simulink model "dual_thyristor_bridge_rectifier"  (R2025b)
settings: Solver=ode1be  StartTime=0.0  StopTime=simlength  FixedStep=tc  MaxStep=tc
values from neighbouring files (symbols this model uses):
  n1 = 35    [voltage_spectrum_analysis.m]
  omega_grid_emulator_nom = w_grid    (= 314.159265359)    [grid_emulator.m]
  vn_eta_pu = 0    [grid_emulator.m]
  vn_xi_pu = 0    [grid_emulator.m]
  vp_xi_pu = 1    [grid_emulator.m]
  w_grid = f_grid*2*pi    (= 314.159265359)    [grid_emulator.m]
undefined symbols (not defined in the file or in its folder): CSF_11, CSF_13, CSF_5, CSF_7, delta_fht1, Idc_traction_normalization_factor, ki_u_ctrl, kp_u_ctrl, Ld_fht1, LFu_dc, LSF_11, LSF_13, LSF_5, LSF_7, magnitude, n10, omega_fht1, pll_i1, pll_p, RLFu_dc, tc, Tcontrol_rect, ts_ctrl_rect, ugrid_factor, Vdc_traction_normalization_factor, Vgrid_phase_normalization_factor
libraries: fl_lib x299, nesl_utility x67, ee_lib x24, single_phase_transformer_lib x3, cstblocks x3
(part 1 of 6)
settings Model: SimulationMode=accelerator  Creator=dbagn  LastModifiedBy=ltnbda
settings SolverCC: NumberNewtonIterations=3.0  ZeroCrossControl=DisableAll  AlgebraicLoopSolver=TrustRegion  SolverResetMethod=Robust
settings DataIOCC: SaveOutput=off  SignalLogging=off  DSMLogging=off  SaveTime=off  ReturnWorkspaceOutputs=off
settings OptimizationCC: ReuseModelBlockBuffer=off  SimCompilerOptimization=on
settings DebuggingCC: UnconnectedInputMsg=warning  UnconnectedOutputMsg=warning  UnconnectedLineMsg=warning
settings ModelReferenceCC: EnableRefExpFcnMdlSchedulingChecks=on
settings SFSimCC: CustomCodeUndefinedFunction=ThrowError
settings SFSimCC: SimCustomHeaderCode=|
  | #include "math_f.h"
  | #include "mavgflt.h"
  | #include "mavgflt_simulink.h"
  | #include "bemf_obsv.h"
  | #include "bemf_obsv_simulink.h"
  | #include "bemf_obsv_load_est.h"
  | #include "bemf_obsv_load_est_simulink.h"
  | #include "dqvector_pi.h"
  | #include "dqvector_pi_simulink.h"
  | #include "sv_pwm_simulink.h"
  | #include "sv_pwm.h"
  | #include "twelve_pulse_rect.h"
  | #include "first_harmonic_tracker.h"
  | #include "first_harmonic_tracker_simulink.h"
  | #include "dqpll_thyr.h"
  | #include "dqpll_thyr_simulink.h"
  | #include "dqpll_grid.h"
  | #include "dqpll_grid_simulink.h"
settings SFSimCC: SimUserSources=|
  | "mavgflt_simulink.c"
  | "mavgflt.c"
  | "bemf_obsv_simulink.c"
  | "bemf_obsv.c"
  | "bemf_obsv_load_est_simulink.c"
  | "bemf_obsv_load_est.c"
  | "dqvector_pi.c"
  | "dqvector_pi_simulink.c"
  | "sv_pwm_simulink.c"
  | "sv_pwm.c"
  | "twelve_pulse_rect.c"
  | "first_harmonic_tracker_simulink.c"
  | "first_harmonic_tracker.c"
  | "dqpll_thyr_simulink.c"
  | "dqpll_thyr.c"
  | "dqpll_grid_simulink.c"
  | "dqpll_grid.c"
settings SFSimCC: SimUserIncludeDirs=|
  | include
  | src
settings RTWCC: GPUComputeCapability=3.5  DLArmComputeVersion=19.05

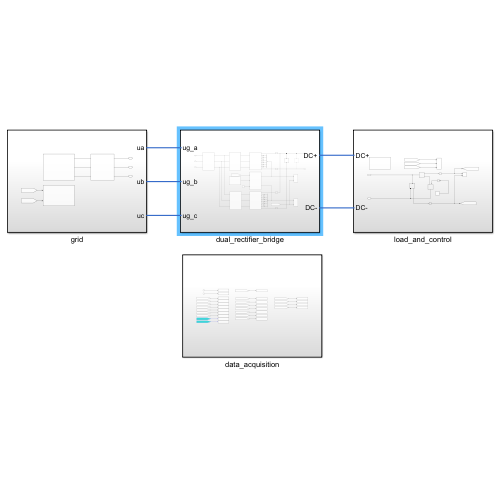
[thumbnail: Simulink's stored preview of the top-level diagram]
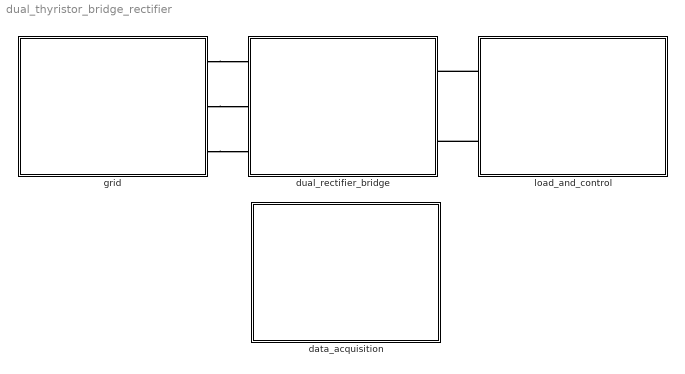
== system dual_thyristor_bridge_rectifier ==
  data_acquisition : Subsystem
  dual_rectifier_bridge : Subsystem
  grid : Subsystem
  load_and_control : Subsystem
  connections:
  grid/RConn1 -- dual_rectifier_bridge/LConn1
  grid/RConn2 -- dual_rectifier_bridge/LConn2
  grid/RConn3 -- dual_rectifier_bridge/LConn3
  load_and_control/LConn1 -- dual_rectifier_bridge/RConn1
  load_and_control/LConn2 -- dual_rectifier_bridge/RConn2

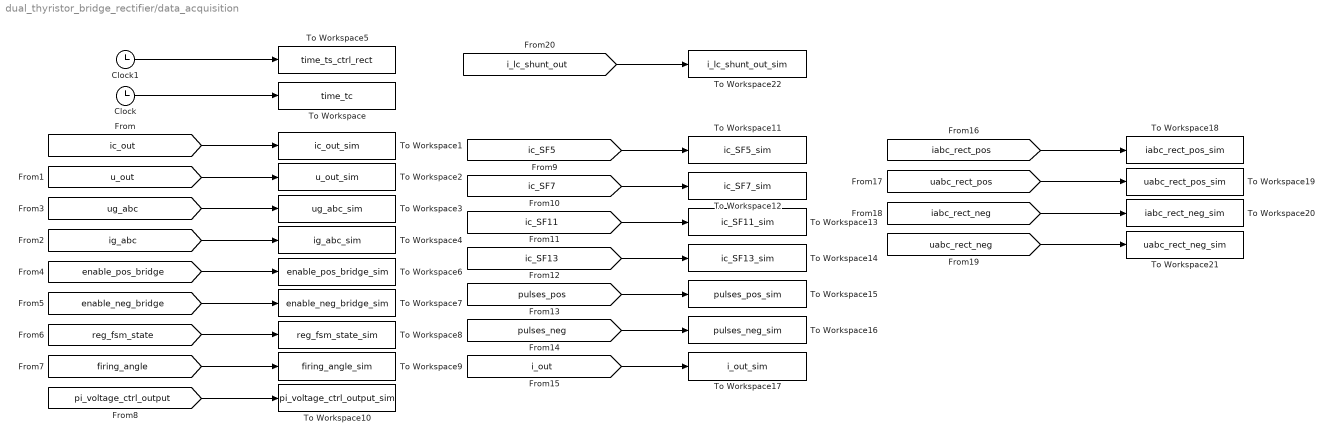
== system dual_thyristor_bridge_rectifier/data_acquisition ==
  Clock : Clock
  Clock1 : Clock
  To Workspace : ToWorkspace  VariableName=time_tc  SaveFormat=Timeseries  SampleTime=tc
      settings: MaxDataPoints=Nc
  To Workspace1 : ToWorkspace  VariableName=ic_out_sim  SaveFormat=Timeseries  SampleTime=tc
      settings: MaxDataPoints=Nc
  To Workspace10 : ToWorkspace  VariableName=pi_voltage_ctrl_output_sim  SaveFormat=Timeseries  SampleTime=ts_ctrl_rect
      settings: MaxDataPoints=Ns_ctrl_rect
  To Workspace11 : ToWorkspace  VariableName=ic_SF5_sim  SaveFormat=Timeseries  SampleTime=tc
      settings: MaxDataPoints=Nc
  To Workspace12 : ToWorkspace  VariableName=ic_SF7_sim  SaveFormat=Timeseries  SampleTime=tc
      settings: MaxDataPoints=Nc
  To Workspace13 : ToWorkspace  VariableName=ic_SF11_sim  SaveFormat=Timeseries  SampleTime=tc
      settings: MaxDataPoints=Nc
  To Workspace14 : ToWorkspace  VariableName=ic_SF13_sim  SaveFormat=Timeseries  SampleTime=tc
      settings: MaxDataPoints=Nc
  To Workspace15 : ToWorkspace  VariableName=pulses_pos_sim  SaveFormat=Timeseries  SampleTime=tc
      settings: MaxDataPoints=Nc
  To Workspace16 : ToWorkspace  VariableName=pulses_neg_sim  SaveFormat=Timeseries  SampleTime=tc
      settings: MaxDataPoints=Nc
  To Workspace17 : ToWorkspace  VariableName=i_out_sim  SaveFormat=Timeseries  SampleTime=tc
      settings: MaxDataPoints=Nc
  To Workspace18 : ToWorkspace  VariableName=iabc_rect_pos_sim  SaveFormat=Timeseries  SampleTime=tc
      settings: MaxDataPoints=Nc
  To Workspace19 : ToWorkspace  VariableName=uabc_rect_pos_sim  SaveFormat=Timeseries  SampleTime=tc
      settings: MaxDataPoints=Nc
  To Workspace2 : ToWorkspace  VariableName=u_out_sim  SaveFormat=Timeseries  SampleTime=tc
      settings: MaxDataPoints=Nc
  To Workspace20 : ToWorkspace  VariableName=iabc_rect_neg_sim  SaveFormat=Timeseries  SampleTime=tc
      settings: MaxDataPoints=Nc
  To Workspace21 : ToWorkspace  VariableName=uabc_rect_neg_sim  SaveFormat=Timeseries  SampleTime=tc
      settings: MaxDataPoints=Nc
  To Workspace22 : ToWorkspace  VariableName=i_lc_shunt_out_sim  SaveFormat=Timeseries  SampleTime=tc
      settings: MaxDataPoints=Nc
  To Workspace3 : ToWorkspace  VariableName=ug_abc_sim  SaveFormat=Timeseries  SampleTime=tc
      settings: MaxDataPoints=Nc
  To Workspace4 : ToWorkspace  VariableName=ig_abc_sim  SaveFormat=Timeseries  SampleTime=tc
      settings: MaxDataPoints=Nc
  To Workspace5 : ToWorkspace  VariableName=time_ts_ctrl_rect  SaveFormat=Timeseries  SampleTime=tc
      settings: MaxDataPoints=Nc
  To Workspace6 : ToWorkspace  VariableName=enable_pos_bridge_sim  SaveFormat=Timeseries  SampleTime=ts_ctrl_rect
      settings: MaxDataPoints=Ns_ctrl_rect
  To Workspace7 : ToWorkspace  VariableName=enable_neg_bridge_sim  SaveFormat=Timeseries  SampleTime=ts_ctrl_rect
      settings: MaxDataPoints=Ns_ctrl_rect
  To Workspace8 : ToWorkspace  VariableName=reg_fsm_state_sim  SaveFormat=Timeseries  SampleTime=ts_ctrl_rect
      settings: MaxDataPoints=Ns_ctrl_rect
  To Workspace9 : ToWorkspace  VariableName=firing_angle_sim  SaveFormat=Timeseries  SampleTime=ts_ctrl_rect
      settings: MaxDataPoints=Ns_ctrl_rect
  wires:
  [ic_out] -> To Workspace1/1
  Clock/1 -> To Workspace/1
  [ug_abc] -> To Workspace3/1
  [ig_abc] -> To Workspace4/1
  [u_out] -> To Workspace2/1
  Clock1/1 -> To Workspace5/1
  [enable_pos_bridge] -> To Workspace6/1
  [enable_neg_bridge] -> To Workspace7/1
  [reg_fsm_state] -> To Workspace8/1
  [firing_angle] -> To Workspace9/1
  [pi_voltage_ctrl_output] -> To Workspace10/1
  [ic_SF5] -> To Workspace11/1
  [ic_SF7] -> To Workspace12/1
  [ic_SF11] -> To Workspace13/1
  [ic_SF13] -> To Workspace14/1
  [pulses_pos] -> To Workspace15/1
  [pulses_neg] -> To Workspace16/1
  [i_out] -> To Workspace17/1
  [iabc_rect_pos] -> To Workspace18/1
  [uabc_rect_pos] -> To Workspace19/1
  [uabc_rect_neg] -> To Workspace21/1
  [iabc_rect_neg] -> To Workspace20/1
  [i_lc_shunt_out] -> To Workspace22/1

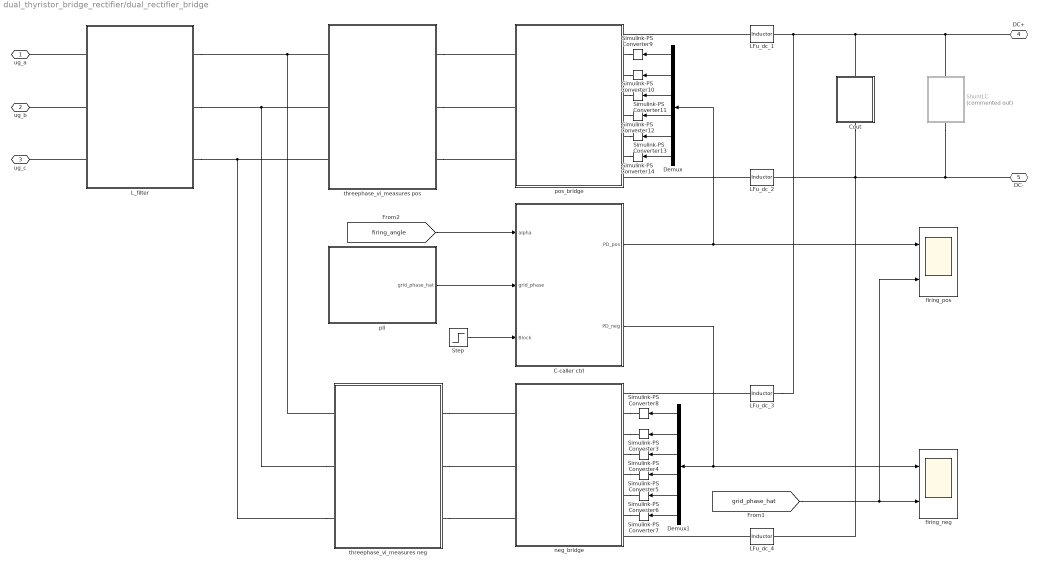
== system dual_thyristor_bridge_rectifier/dual_rectifier_bridge ==
  C-caller ctrl : Subsystem
  Cout : Subsystem
  Demux : Demux  Outputs=6
  Demux1 : Demux  Outputs=6
  LFu_dc_{1..4} (4 alike) : fl_lib/Electrical/Electrical Elements/Inductor  l=LFu_dc/2 H  r=RLFu_dc/2 Ohm  g=1e-9 1/Ohm  i_specify=off  i_priority=None  i=0 A  i_nominal_specify=off  i_nominal_value=1  i_nominal_unit=A  v_specify=off  v_priority=None  v=0 V  v_nominal_specify=off  v_nominal_value=1  v_nominal_unit=V  i_L_specify=off  i_L_priority=High  i_L=0 A  i_L_nominal_specify=off  i_L_nominal_value=1  i_L_nominal_unit=A
  L_filter : Subsystem
  ShuntLC : Subsystem  Commented=on
  Simulink-PS Converter{3,5..10,12..14} (10 alike) : nesl_utility/Simulink-PS Converter  PhysicalDomain=network_engine_domain  SubClassName=ps_input  LeftPortType=input  RightPortType=output  PseudoPeriodic=off  Frequencies=[]  NoiseDistribution=none  NoiseParameters=[]  Unit=V  AffineConversion=on  FilteringAndDerivatives=provide  SimscapeFilterOrder=1  InputFilterTimeConstant=0.001  UdotUserProvided=0
  Simulink-PS Converter11 : nesl_utility/Simulink-PS Converter  PhysicalDomain=network_engine_domain  SubClassName=ps_input  LeftPortType=input  RightPortType=output  PseudoPeriodic=off  Frequencies=[]  NoiseDistribution=none  NoiseParameters=[]  Unit=V  AffineConversion=off  FilteringAndDerivatives=provide  SimscapeFilterOrder=1  InputFilterTimeConstant=0.001  UdotUserProvided=0
  Simulink-PS Converter4 : nesl_utility/Simulink-PS Converter  PhysicalDomain=network_engine_domain  SubClassName=ps_input  LeftPortType=input  RightPortType=output  PseudoPeriodic=off  Frequencies=[]  NoiseDistribution=none  NoiseParameters=[]  Unit=V  AffineConversion=off  FilteringAndDerivatives=provide  SimscapeFilterOrder=1  InputFilterTimeConstant=0.001  UdotUserProvided=0
  Step : Step  Time=0  Before=1  After=0
  firing_neg : Scope  NumInputPorts=2
      settings: SampleTime=ts  ActiveDisplayYMinimum=-1.5  ActiveDisplayYMaximum=13.5
  firing_pos : Scope  NumInputPorts=2
      settings: SampleTime=ts  ActiveDisplayYMinimum=-1.5  ActiveDisplayYMaximum=13.5
  neg_bridge : Subsystem
  pll : Subsystem
  pos_bridge : Subsystem
  threephase_vi_measures neg : Subsystem
  threephase_vi_measures pos : Subsystem
  ug_a : PMIOPort  Side=Left
  ug_b : PMIOPort  Port=2  Side=Left
  ug_c : PMIOPort  Port=3  Side=Left
  DC+ : PMIOPort  Port=4  Side=Right
  DC- : PMIOPort  Port=5  Side=Right
  wires:
  Demux1/1 -> Simulink-PS Converter8/1
  Step/1 -> C-caller ctrl/3(Block)
  C-caller ctrl/1(PD_pos) -> firing_pos/1, Demux/1
  Demux/6 -> Simulink-PS Converter14/1
  Demux1/4 -> Simulink-PS Converter5/1
  Demux1/6 -> Simulink-PS Converter7/1
  [firing_angle] -> C-caller ctrl/1(alpha)
  Demux1/3 -> Simulink-PS Converter4/1
  Demux/4 -> Simulink-PS Converter12/1
  pll/1(grid_phase_hat) -> C-caller ctrl/2(grid_phase)
  C-caller ctrl/2(PD_neg) -> firing_neg/1, Demux1/1
  Demux1/2 -> Simulink-PS Converter3/1
  Demux/1 -> Simulink-PS Converter9/1
  Demux/2 -> Simulink-PS Converter10/1
  Demux/3 -> Simulink-PS Converter11/1
  Demux1/5 -> Simulink-PS Converter6/1
  Demux/5 -> Simulink-PS Converter13/1
  [grid_phase_hat] -> firing_neg/2, firing_pos/2
  connections:
  L_filter/RConn1 -- ug_a/RConn1
  L_filter/RConn2 -- ug_b/RConn1
  L_filter/RConn3 -- ug_c/RConn1
  pos_bridge/LConn3 -- Simulink-PS Converter10/RConn1
  neg_bridge/LConn6 -- Simulink-PS Converter6/RConn1
  neg_bridge/LConn5 -- Simulink-PS Converter5/RConn1
  pos_bridge/LConn5 -- Simulink-PS Converter12/RConn1
  neg_bridge/LConn2 -- Simulink-PS Converter8/RConn1
  pos_bridge/LConn2 -- Simulink-PS Converter9/RConn1
  neg_bridge/LConn3 -- Simulink-PS Converter3/RConn1
  pos_bridge/LConn4 -- Simulink-PS Converter11/RConn1
  neg_bridge/LConn7 -- Simulink-PS Converter7/RConn1
  pos_bridge/LConn6 -- Simulink-PS Converter13/RConn1
  pos_bridge/LConn7 -- Simulink-PS Converter14/RConn1
  neg_bridge/LConn4 -- Simulink-PS Converter4/RConn1
  threephase_vi_measures neg/LConn2 -- L_filter/LConn2 -- threephase_vi_measures pos/LConn2
  L_filter/LConn1 -- threephase_vi_measures neg/LConn1 -- threephase_vi_measures pos/LConn1
  threephase_vi_measures neg/LConn3 -- L_filter/LConn3 -- threephase_vi_measures pos/LConn3
  threephase_vi_measures pos/RConn1 -- pos_bridge/RConn1
  threephase_vi_measures pos/RConn2 -- pos_bridge/RConn2
  threephase_vi_measures pos/RConn3 -- pos_bridge/RConn3
  threephase_vi_measures neg/RConn1 -- neg_bridge/RConn1
  threephase_vi_measures neg/RConn2 -- neg_bridge/RConn2
  threephase_vi_measures neg/RConn3 -- neg_bridge/RConn3
  LFu_dc_4/RConn1 -- LFu_dc_2/RConn1 -- Cout/RConn1 -- ShuntLC/RConn1 -- DC-/RConn1
  LFu_dc_1/RConn1 -- LFu_dc_3/RConn1 -- Cout/LConn1 -- ShuntLC/LConn1 -- DC+/RConn1
  LFu_dc_1/LConn1 -- pos_bridge/LConn1
  LFu_dc_2/LConn1 -- pos_bridge/LConn8
  neg_bridge/LConn1 -- LFu_dc_3/LConn1
  LFu_dc_4/LConn1 -- neg_bridge/LConn8

== system dual_thyristor_bridge_rectifier/grid ==
  grid_emulator : Subsystem
  instantaneus_power : Subsystem
  threephase_vi_measures : Subsystem
  ua : PMIOPort  Side=Right
  ub : PMIOPort  Port=2  Side=Right
  uc : PMIOPort  Port=3  Side=Right
  wires:
  [ug_abc] -> instantaneus_power/1(Vline)
  [ig_abc] -> instantaneus_power/2(Iline)
  connections:
  threephase_vi_measures/LConn3 -- grid_emulator/RConn3
  threephase_vi_measures/LConn1 -- grid_emulator/RConn1
  threephase_vi_measures/RConn2 -- ub/RConn1
  threephase_vi_measures/LConn2 -- grid_emulator/RConn2
  threephase_vi_measures/RConn1 -- ua/RConn1
  threephase_vi_measures/RConn3 -- uc/RConn1

== system dual_thyristor_bridge_rectifier/load_and_control ==
  Controlled Current Source : fl_lib/Electrical/Electrical Sources/Controlled Current Source
  Current Sensor : fl_lib/Electrical/Electrical Sensors/Current Sensor
  PS-Simulink Converter : nesl_utility/PS-Simulink Converter  PhysicalDomain=network_engine_domain  SubClassName=ps_output  LeftPortType=input  RightPortType=output  PseudoPeriodic=off  Frequencies=[]  VectorFormat=1-D array  Unit=A  AffineConversion=off
  PS-Simulink Converter1 : nesl_utility/PS-Simulink Converter  PhysicalDomain=network_engine_domain  SubClassName=ps_output  LeftPortType=input  RightPortType=output  PseudoPeriodic=off  Frequencies=[]  VectorFormat=1-D array  Unit=V  AffineConversion=on
  Simulink-PS Converter : nesl_utility/Simulink-PS Converter  PhysicalDomain=network_engine_domain  SubClassName=ps_input  LeftPortType=input  RightPortType=output  PseudoPeriodic=off  Frequencies=[]  NoiseDistribution=none  NoiseParameters=[]  Unit=1  AffineConversion=off  FilteringAndDerivatives=provide  SimscapeFilterOrder=1  InputFilterTimeConstant=0.001  UdotUserProvided=0
  Sine Wave : Sin  Amplitude=Idc_traction_normalization_factor  Frequency=pi/2  SampleTime=0
  Voltage Sensor : fl_lib/Electrical/Electrical Sensors/Voltage Sensor
  controller : Subsystem
  iu_out : Scope  NumInputPorts=2
      settings: SampleTime=ts  ActiveDisplayYMinimum=-2016.1290322580644  ActiveDisplayYMaximum=2016.1290322580644  DataLoggingVariableName=ScopeData3
  ui_Cout : Scope  NumInputPorts=3
      settings: SampleTime=ts  ActiveDisplayYMinimum=-646.93724  ActiveDisplayYMaximum=1108.66938
  DC+ : PMIOPort  Side=Left
  DC- : PMIOPort  Port=2  Side=Left
  tag scope: i_out=global, u_out=global
  wires:
  PS-Simulink Converter/1 -> [i_out], iu_out/1  "i_out"
  PS-Simulink Converter1/1 -> [u_out], iu_out/2  "u_out"
  Sine Wave/1 -> Simulink-PS Converter/1
  [u_out] -> ui_Cout/2  "u_out"
  [ic_out] -> ui_Cout/1  "ic_out"
  [i_lc_shunt_out] -> ui_Cout/3  "i_lc_shunt_out"
  connections:
  Voltage Sensor/RConn1 -- PS-Simulink Converter1/LConn1
  DC+/RConn1 -- Current Sensor/LConn1 -- Voltage Sensor/LConn1
  Simulink-PS Converter/RConn1 -- Controlled Current Source/RConn1
  Current Sensor/RConn2 -- Controlled Current Source/RConn2
  PS-Simulink Converter/LConn1 -- Current Sensor/RConn1
  DC-/RConn1 -- Controlled Current Source/LConn1 -- Voltage Sensor/RConn2

== system dual_thyristor_bridge_rectifier/dual_rectifier_bridge/C-caller ctrl ==
  alpha : Inport
  grid_phase : Inport  Port=2
  Block : Inport  Port=3
  C Caller : CCaller  FunctionName=twvprProcessSimulink  PortSpecificationStruct="%)30     .    R @   8    (     @         %    \"     4    !     0         %  0 \"0    $    _    07)G3F%M90  4&]R=$YA;64 4V-O<&4     26YD97@     5'EP90      4VEZ90      27-';&]B86P   X    P    !@    @    $          4    (     0    (    !         !   @!W=   #@   #     &    \"     0         !0    @    !     @    $         $  \" '=T   .    .     8    (    !          %    \"     $    %     0         0  ...(+2649 chars)"  SampleTime=ts_ctrl_rect
  Constant : Constant  Value=[0 0 0 0 0 0]
  Data Type Conversion1 : DataTypeConversion  OutDataTypeStr=single  SaturateOnIntegerOverflow=off  RndMeth=Floor
  Data Type Conversion2 : DataTypeConversion  OutDataTypeStr=single  SaturateOnIntegerOverflow=off  RndMeth=Floor
  Data Type Conversion4 : DataTypeConversion  OutDataTypeStr=int32  SaturateOnIntegerOverflow=off  RndMeth=Floor
  Subsystem2 : Subsystem
  Subsystem3 : Subsystem
  Zero-Order Hold1 : ZeroOrderHold  SampleTime=ts_ctrl_rect
  Zero-Order Hold2 : ZeroOrderHold  SampleTime=ts_ctrl_rect
  Zero-Order Hold3 : ZeroOrderHold  SampleTime=ts_ctrl_rect
  neg : Switch  Criteria=u2 > Threshold  Threshold=0.5  SaturateOnIntegerOverflow=off  InputSameDT=off
  pos : Switch  Criteria=u2 > Threshold  Threshold=0.5  SaturateOnIntegerOverflow=off  InputSameDT=off
  PD_pos : Outport  InitialOutput=0  VectorParamsAs1DForOutWhenUnconnected=off
  PD_neg : Outport  Port=2  InitialOutput=0  VectorParamsAs1DForOutWhenUnconnected=off
  tag scope: pulses_neg=global, pulses_pos=global
  wires:
  alpha/1 -> Data Type Conversion2/1
  grid_phase/1 -> Data Type Conversion1/1
  Data Type Conversion2/1 -> Zero-Order Hold2/1
  Data Type Conversion1/1 -> Zero-Order Hold3/1
  Data Type Conversion4/1 -> Zero-Order Hold1/1
  Block/1 -> Data Type Conversion4/1
  C Caller/1 -> Subsystem3/1("PY ")
  C Caller/2 -> Subsystem2/1("PD ")
  Constant/1 -> pos/3, neg/3
  Subsystem2/1(PD) -> neg/1, pos/1
  [enable_pos_bridge] -> pos/2
  [enable_neg_bridge] -> neg/2
  pos/1 -> [pulses_pos], PD_pos/1
  neg/1 -> [pulses_neg], PD_neg/1
  Zero-Order Hold3/1 -> C Caller/1
  Zero-Order Hold2/1 -> C Caller/2
  Zero-Order Hold1/1 -> C Caller/3

== system dual_thyristor_bridge_rectifier/dual_rectifier_bridge/Cout ==
  Capacitor : fl_lib/Electrical/Electrical Elements/Capacitor  c=CFu_dc F  r=RCFu_dc Ohm  g=0 1/Ohm  i_specify=off  i_priority=None  i=0 A  i_nominal_specify=off  i_nominal_value=1  i_nominal_unit=A  v_specify=off  v_priority=None  v=0 V  v_nominal_specify=off  v_nominal_value=1  v_nominal_unit=V  vc_specify=off  vc_priority=High  vc=0 V  vc_nominal_specify=off  vc_nominal_value=1  vc_nominal_unit=V
  Current Sensor1 : fl_lib/Electrical/Electrical Sensors/Current Sensor
  PS-Simulink Converter2 : nesl_utility/PS-Simulink Converter  PhysicalDomain=network_engine_domain  SubClassName=ps_output  LeftPortType=input  RightPortType=output  PseudoPeriodic=off  Frequencies=[]  VectorFormat=1-D array  Unit=A  AffineConversion=off
  u+ : PMIOPort  Side=Left
  u- : PMIOPort  Port=2  Side=Right
  tag scope: ic_out=global
  wires:
  PS-Simulink Converter2/1 -> [ic_out]
  connections:
  Capacitor/RConn1 -- u-/RConn1
  Current Sensor1/RConn2 -- Capacitor/LConn1
  PS-Simulink Converter2/LConn1 -- Current Sensor1/RConn1
  Current Sensor1/LConn1 -- u+/RConn1

== system dual_thyristor_bridge_rectifier/dual_rectifier_bridge/L_filter ==
  Inductor : fl_lib/Electrical/Electrical Elements/Inductor  l=1e-6 H  r=0 Ohm  g=1e-9 1/Ohm  i_specify=on  i_priority=High  i=0 A  i_nominal_specify=off  i_nominal_value=1  i_nominal_unit=A  v_specify=off  v_priority=None  v=0 V  v_nominal_specify=off  v_nominal_value=1  v_nominal_unit=V  i_L_specify=off  i_L_priority=High  i_L=0 A  i_L_nominal_specify=off  i_L_nominal_value=1  i_L_nominal_unit=A
  Inductor1 : fl_lib/Electrical/Electrical Elements/Inductor  l=1e-6 H  r=0 Ohm  g=1e-9 1/Ohm  i_specify=on  i_priority=High  i=0 A  i_nominal_specify=off  i_nominal_value=1  i_nominal_unit=A  v_specify=off  v_priority=None  v=0 V  v_nominal_specify=off  v_nominal_value=1  v_nominal_unit=V  i_L_specify=off  i_L_priority=High  i_L=0 A  i_L_nominal_specify=off  i_L_nominal_value=1  i_L_nominal_unit=A
  Inductor2 : fl_lib/Electrical/Electrical Elements/Inductor  l=1e-6 H  r=0 Ohm  g=1e-9 1/Ohm  i_specify=on  i_priority=High  i=0 A  i_nominal_specify=off  i_nominal_value=1  i_nominal_unit=A  v_specify=off  v_priority=None  v=0 V  v_nominal_specify=off  v_nominal_value=1  v_nominal_unit=V  i_L_specify=off  i_L_priority=High  i_L=0 A  i_L_nominal_specify=off  i_L_nominal_value=1  i_L_nominal_unit=A
  i_SFs : Scope  NumInputPorts=4
      settings: SampleTime=tc  ActiveDisplayYMinimum=-334.41525  ActiveDisplayYMaximum=336.06574  DataLoggingVariableName=ScopeData2
  shunt_passive_filter_11 : Subsystem  mask{CSF=CSF_11, LSF=LSF_11, RCSF=5e-3}
      mask prompts: CSF "Shunt Capacitor"; LSF "Shunt Inductor"; RCSF "Shunt Resistor"
      mask Display: disp('SPF');
  shunt_passive_filter_13 : Subsystem  mask{CSF=CSF_13, LSF=LSF_13, RCSF=5e-3}
      mask prompts: CSF "Shunt Capacitor"; LSF "Shunt Inductor"; RCSF "Shunt Resistor"
      mask Display: disp('SPF');
  shunt_passive_filter_5 : Subsystem  mask{CSF=CSF_5, LSF=LSF_5, RCSF=5e-3}
      mask prompts: CSF "Shunt Capacitor"; LSF "Shunt Inductor"; RCSF "Shunt Resistor"
      mask Display: disp('SPF');
  shunt_passive_filter_7 : Subsystem  mask{CSF=CSF_7, LSF=LSF_7, RCSF=5e-3}
      mask prompts: CSF "Shunt Capacitor"; LSF "Shunt Inductor"; RCSF "Shunt Resistor"
      mask Display: disp('SPF');
  ui_measure : Subsystem
  us_a : PMIOPort  Side=Left
  ug_a : PMIOPort  Port=2  Side=Right
  us_b : PMIOPort  Port=3  Side=Left
  ug_b : PMIOPort  Port=4  Side=Right
  us_c : PMIOPort  Port=5  Side=Left
  ug_c : PMIOPort  Port=6  Side=Right
  wires:
  [ic_SF5] -> i_SFs/1
  [ic_SF7] -> i_SFs/2
  [ic_SF11] -> i_SFs/3
  [ic_SF13] -> i_SFs/4
  connections:
  ui_measure/RConn1 -- shunt_passive_filter_7/RConn1 -- shunt_passive_filter_11/RConn1 -- shunt_passive_filter_13/RConn1 -- Inductor/LConn1 -- shunt_passive_filter_5/RConn1
  ui_measure/RConn2 -- shunt_passive_filter_7/RConn2 -- shunt_passive_filter_11/RConn2 -- shunt_passive_filter_13/RConn2 -- Inductor1/LConn1 -- shunt_passive_filter_5/RConn2
  ui_measure/RConn3 -- shunt_passive_filter_7/RConn3 -- shunt_passive_filter_11/RConn3 -- shunt_passive_filter_13/RConn3 -- Inductor2/LConn1 -- shunt_passive_filter_5/RConn3
  us_a/RConn1 -- Inductor/RConn1
  Inductor1/RConn1 -- us_b/RConn1
  Inductor2/RConn1 -- us_c/RConn1
  ug_b/RConn1 -- ui_measure/LConn2
  ug_a/RConn1 -- ui_measure/LConn1
  ug_c/RConn1 -- ui_measure/LConn3

== system dual_thyristor_bridge_rectifier/dual_rectifier_bridge/ShuntLC ==
  Capacitor : fl_lib/Electrical/Electrical Elements/Capacitor  c=C_shunt_dc F  r=RC_shunt_dc Ohm  g=0 1/Ohm  i_specify=off  i_priority=None  i=0 A  i_nominal_specify=off  i_nominal_value=1  i_nominal_unit=A  v_specify=off  v_priority=None  v=0 V  v_nominal_specify=off  v_nominal_value=1  v_nominal_unit=V  vc_specify=off  vc_priority=High  vc=0 V  vc_nominal_specify=off  vc_nominal_value=1  vc_nominal_unit=V
  Capacitor1 : fl_lib/Electrical/Electrical Elements/Capacitor  c=C_shunt_dc F  r=RC_shunt_dc Ohm  g=0 1/Ohm  i_specify=off  i_priority=None  i=0 A  i_nominal_specify=off  i_nominal_value=1  i_nominal_unit=A  v_specify=off  v_priority=None  v=0 V  v_nominal_specify=off  v_nominal_value=1  v_nominal_unit=V  vc_specify=off  vc_priority=High  vc=0 V  vc_nominal_specify=off  vc_nominal_value=1  vc_nominal_unit=V
  Current Sensor1 : fl_lib/Electrical/Electrical Sensors/Current Sensor
  Inductor : fl_lib/Electrical/Electrical Elements/Inductor  l=L_shunt_dc H  r=0 Ohm  g=1e-9 1/Ohm  i_specify=off  i_priority=None  i=0 A  i_nominal_specify=off  i_nominal_value=1  i_nominal_unit=A  v_specify=off  v_priority=None  v=0 V  v_nominal_specify=off  v_nominal_value=1  v_nominal_unit=V  i_L_specify=off  i_L_priority=High  i_L=0 A  i_L_nominal_specify=off  i_L_nominal_value=1  i_L_nominal_unit=A
  PS-Simulink Converter2 : nesl_utility/PS-Simulink Converter  PhysicalDomain=network_engine_domain  SubClassName=ps_output  LeftPortType=input  RightPortType=output  PseudoPeriodic=off  Frequencies=[]  VectorFormat=1-D array  Unit=A  AffineConversion=off
  u+ : PMIOPort  Side=Left
  u- : PMIOPort  Port=2  Side=Right
  tag scope: i_lc_shunt_out=global
  wires:
  PS-Simulink Converter2/1 -> [i_lc_shunt_out]
  connections:
  Current Sensor1/LConn1 -- u+/RConn1
  PS-Simulink Converter2/LConn1 -- Current Sensor1/RConn1
  Current Sensor1/RConn2 -- Capacitor1/LConn1 -- Capacitor/LConn1
  Capacitor/RConn1 -- Capacitor1/RConn1 -- Inductor/LConn1
  Inductor/RConn1 -- u-/RConn1

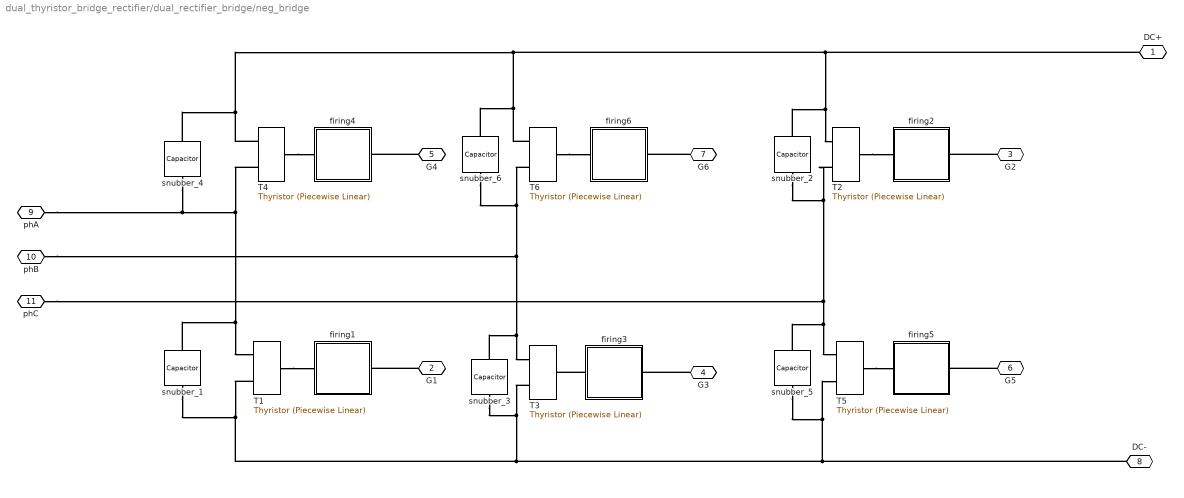
== system dual_thyristor_bridge_rectifier/dual_rectifier_bridge/neg_bridge ==
  T{1..6} (6 alike) : ee_lib/Semiconductors & Converters/Thyristor (Piecewise Linear)  port_option=ee.enum.controlport.ps  Vf=0.8 V  Ron=0.001 Ohm  Goff=1e-5 1/Ohm  Vgt=6 V  Ih=1 A  diode_param=1  diode_Vf=0.8 V  diode_Ron=0.001 Ohm  diode_Goff=1e-5 1/Ohm  diode_C=50e-9 F  diode_iRM=-235 A  diode_iF=300 A  diode_idot=-50 A/us  diode_trr_param=1  diode_trr_factor=3  diode_trr=15 us  diode_Qrr=1500 s*uA  iak_specify=off  iak_priority=None  iak=0 A  iak_nominal_specify=off  iak_nominal_value=1  iak_nominal_unit=A  vak_specify=off  vak_priority=None  vak=0 V  vak_nominal_specify=off  vak_nominal_value=1  vak_nominal_unit=V  vgk_specify=off  vgk_priority=None  vgk=0 V  vgk_nominal_specify=off  vgk_nominal_value=1  vgk_nominal_unit=V  thermal_loss_option=2  Von_data=[0, 1.1, 1.3, 1.45, 1.75, 2.25, 2.7; 0, 1, 1.15, 1.35, 1.7, 2.35, 3] V  Tj=[298.15, 398.15] K  Iout_data=[0, 10, 50, 100, 200, 400, 600] A  Eon_data=[0, .29, 1.43, 2.86, 5.71, 13.14, 22.86; 0, .57, 2.63, 5.14, 10.29, 20.57, 30.29] * 1e-3 J  Tj_loss=[298.15, 398.15] K  Iout_data_loss=[0, .1, 1, 5, 10, 20, 40, 70, 100] A  Eon_scalar=22.86e-3 J  Eoff_natural_commutation=10e-3 J  Voff=300 V  Iout_scalar=600 A  onCurrentMeasDelay=1e-4 s  diodeModelType=ee.enum.converters.diodeModelType.pwl  diodeTableType=ee.enum.diode.tableType.IfMat  diode_IfMat=[.07, .12, .19, 1.75, 4.24, 7.32, 11.2; .16, .3, .72, 2.14, 4.02, 6.35, 9.12] A  diode_VfMat=[.9, 1.15, 1.25, 1.5, 1.75, 2.17, 2.6, 2.85; .58, .68, .75, 1.1, 1.38, 1.77, 2.27, 2.7] V  diode_TjVec=[25, 125] degC  diode_VfVec=[.5, .7, .9, 1.3, 1.7, 2.1, 2.5] V  diode_IfVec=[.1, .2, .5, 1, 2, 4, 7, 10] A  diode_rec_loss_model=ee.enum.diode.reverseRecoveryModel.fixed  diode_ErecVal=0 J  diode_scaleWithIandV=true  diode_ErecMat=zeros(2, 3) J  diode_TjrecVec=[298.15, 398.15] K  diode_IfrecVec=[.1, 1, 10] A  diode_IrecVal=10 A  diode_VrecVal=10 V  diode_tFilter=1 / 1000 / 100 s  thermal_network_parameterization=ee.enum.thermalNetworkTopology.external  Rth=[.08, .5] K/W  Rth_Cauer=[.08, .1, .5] K/W  Rth_Foster=[.08, .14, .22, .16] K/W  thermal_mass_parameterization=ee.enum.thermalNetwork.timeconstant  thermal_mass=[.01, .5] J/K  thermal_mass_Cauer=[.01, .1, .5] J/K  thermal_mass_Foster=[.001, .005, .05, .5] J/K  thermal_time_constant=[.001, .2] s  thermal_time_constant_Cauer=[.001, .1, .2] s  thermal_time_constant_Foster=[7e-05, .0007, .01, .08] s  thermal_mass_initial_temperatures=[25, 25] degC  thermal_mass_initial_temperatures_Cauer=[25, 25, 25] degC  junction_thermal_mass=0.01 J/K  Tvec_initial_Foster=[25, 25, 25, 25] degC  junction_temperature_specify=off  junction_temperature_priority=None  junction_temperature=25 degC  junction_temperature_nominal_specify=off  junction_temperature_nominal_value=1  junction_temperature_nominal_unit=degC  Qj_specify=off  Qj_priority=None  Qj=0 W  Qj_nominal_specify=off  Qj_nominal_value=1  Qj_nominal_unit=W  accumulatedSwitchingLosses_specify=off  accumulatedSwitchingLosses_priority=None  accumulatedSwitchingLosses=0 J
      settings: InternalSimscapePortConfiguration="{\"Bottom\":[],\"Left\":[{\"id\":\"G\",\"label\":\"\",\"type\":\"input\"}],\"Right\":[{\"id\":\"A\",\"label\":\"\",\"type\":\"foundation.electrical.electrical\"},{\"id\":\"K\",\"label\":\"\",\"type\":\"foundation.electrical.electrical\"}],\"Top\":[]}"
  firing1 : Subsystem
  firing2 : Subsystem
  firing3 : Subsystem
  firing4 : Subsystem
  firing5 : Subsystem
  firing6 : Subsystem
  snubber_{1..6} (6 alike) : fl_lib/Electrical/Electrical Elements/Capacitor  c=Csnubber_scr F  r=Rsnubber_scr Ohm  g=0 1/Ohm  i_specify=off  i_priority=None  i=0 A  i_nominal_specify=off  i_nominal_value=1  i_nominal_unit=A  v_specify=off  v_priority=None  v=0 V  v_nominal_specify=off  v_nominal_value=1  v_nominal_unit=V  vc_specify=off  vc_priority=High  vc=0 V  vc_nominal_specify=off  vc_nominal_value=1  vc_nominal_unit=V
  DC+ : PMIOPort  Side=Left
  G1 : PMIOPort  Port=2  Side=Left
  G2 : PMIOPort  Port=3  Side=Left
  G3 : PMIOPort  Port=4  Side=Left
  G4 : PMIOPort  Port=5  Side=Left
  G5 : PMIOPort  Port=6  Side=Left
  G6 : PMIOPort  Port=7  Side=Left
  DC- : PMIOPort  Port=8  Side=Left
  phA : PMIOPort  Port=9  Side=Right
  phB : PMIOPort  Port=10  Side=Right
  phC : PMIOPort  Port=11  Side=Right
  connections:
  phB/RConn1 -- snubber_6/RConn1 -- T6/RConn2 -- snubber_3/LConn1 -- T3/RConn1
  phC/RConn1 -- snubber_2/RConn1 -- T2/RConn2 -- snubber_5/LConn1 -- T5/RConn1
  snubber_1/RConn1 -- T1/RConn2 -- snubber_3/RConn1 -- T3/RConn2 -- DC-/RConn1 -- snubber_5/RConn1 -- T5/RConn2
  phA/RConn1 -- snubber_4/RConn1 -- snubber_1/LConn1 -- T1/RConn1 -- T4/RConn2
  T6/LConn1 -- firing6/RConn1
  T5/LConn1 -- firing5/RConn1
  T4/LConn1 -- firing4/RConn1
  firing3/RConn1 -- T3/LConn1
  T2/LConn1 -- firing2/RConn1
  T1/LConn1 -- firing1/RConn1
  G6/RConn1 -- firing6/LConn1
  G5/RConn1 -- firing5/LConn1
  G4/RConn1 -- firing4/LConn1
  G3/RConn1 -- firing3/LConn1
  G2/RConn1 -- firing2/LConn1
  G1/RConn1 -- firing1/LConn1
  T4/RConn1 -- snubber_4/LConn1 -- DC+/RConn1 -- snubber_2/LConn1 -- T2/RConn1 -- snubber_6/LConn1 -- T6/RConn1

== system dual_thyristor_bridge_rectifier/dual_rectifier_bridge/pll ==
  Bus Creator : BusCreator  Inputs=2
  grid_phase_hats : Scope
      settings: ActiveDisplayYMinimum=-0.78537  ActiveDisplayYMaximum=7.06836  DataLoggingVariableName=ScopeData2
  pll_stageA : Subsystem
  pll_stageB : Subsystem
  pll_stageB_Ccaller : Subsystem
  grid_phase_hat : Outport
  tag scope: grid_phase_hat=global
  wires:
  pll_stageA/1(Vgrid_a) -> pll_stageB/1(Vgrid_a)
  pll_stageA/2(Vgrid_b) -> pll_stageB/2(Vgrid_b)
  [ug_abc_pll] -> pll_stageA/1(ug)
  pll_stageB/1(wt_grid) -> Bus Creator/2  "grid_phase_hat_ccaller"
  Bus Creator/1 -> grid_phase_hats/1
  pll_stageB_Ccaller/2(gamma_hat) -> [grid_phase_hat], Bus Creator/1, grid_phase_hat/1  "grid_phase_hat_ccaller"

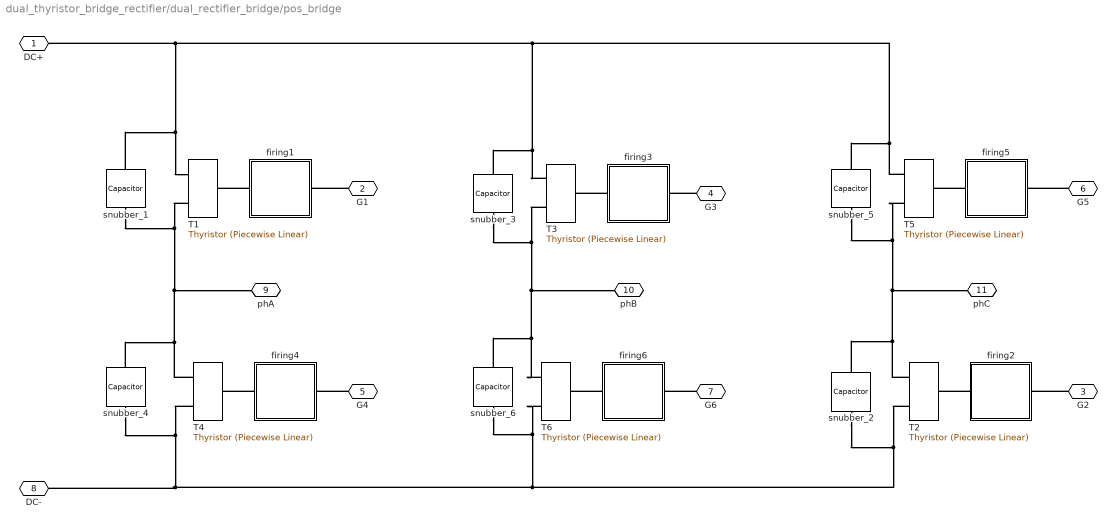
== system dual_thyristor_bridge_rectifier/dual_rectifier_bridge/pos_bridge ==
  T{1..6} (6 alike) : ee_lib/Semiconductors & Converters/Thyristor (Piecewise Linear)  port_option=ee.enum.controlport.ps  Vf=0.8 V  Ron=0.001 Ohm  Goff=1e-5 1/Ohm  Vgt=6 V  Ih=1 A  diode_param=1  diode_Vf=0.8 V  diode_Ron=0.001 Ohm  diode_Goff=1e-5 1/Ohm  diode_C=50e-9 F  diode_iRM=-235 A  diode_iF=300 A  diode_idot=-50 A/us  diode_trr_param=1  diode_trr_factor=3  diode_trr=15 us  diode_Qrr=1500 s*uA  iak_specify=off  iak_priority=None  iak=0 A  iak_nominal_specify=off  iak_nominal_value=1  iak_nominal_unit=A  vak_specify=off  vak_priority=None  vak=0 V  vak_nominal_specify=off  vak_nominal_value=1  vak_nominal_unit=V  vgk_specify=off  vgk_priority=None  vgk=0 V  vgk_nominal_specify=off  vgk_nominal_value=1  vgk_nominal_unit=V  thermal_loss_option=2  Von_data=[0, 1.1, 1.3, 1.45, 1.75, 2.25, 2.7; 0, 1, 1.15, 1.35, 1.7, 2.35, 3] V  Tj=[298.15, 398.15] K  Iout_data=[0, 10, 50, 100, 200, 400, 600] A  Eon_data=[0, .29, 1.43, 2.86, 5.71, 13.14, 22.86; 0, .57, 2.63, 5.14, 10.29, 20.57, 30.29] * 1e-3 J  Tj_loss=[298.15, 398.15] K  Iout_data_loss=[0, .1, 1, 5, 10, 20, 40, 70, 100] A  Eon_scalar=22.86e-3 J  Eoff_natural_commutation=10e-3 J  Voff=300 V  Iout_scalar=600 A  onCurrentMeasDelay=1e-4 s  diodeModelType=ee.enum.converters.diodeModelType.pwl  diodeTableType=ee.enum.diode.tableType.IfMat  diode_IfMat=[.07, .12, .19, 1.75, 4.24, 7.32, 11.2; .16, .3, .72, 2.14, 4.02, 6.35, 9.12] A  diode_VfMat=[.9, 1.15, 1.25, 1.5, 1.75, 2.17, 2.6, 2.85; .58, .68, .75, 1.1, 1.38, 1.77, 2.27, 2.7] V  diode_TjVec=[25, 125] degC  diode_VfVec=[.5, .7, .9, 1.3, 1.7, 2.1, 2.5] V  diode_IfVec=[.1, .2, .5, 1, 2, 4, 7, 10] A  diode_rec_loss_model=ee.enum.diode.reverseRecoveryModel.fixed  diode_ErecVal=0 J  diode_scaleWithIandV=true  diode_ErecMat=zeros(2, 3) J  diode_TjrecVec=[298.15, 398.15] K  diode_IfrecVec=[.1, 1, 10] A  diode_IrecVal=10 A  diode_VrecVal=10 V  diode_tFilter=1 / 1000 / 100 s  thermal_network_parameterization=ee.enum.thermalNetworkTopology.external  Rth=[.08, .5] K/W  Rth_Cauer=[.08, .1, .5] K/W  Rth_Foster=[.08, .14, .22, .16] K/W  thermal_mass_parameterization=ee.enum.thermalNetwork.timeconstant  thermal_mass=[.01, .5] J/K  thermal_mass_Cauer=[.01, .1, .5] J/K  thermal_mass_Foster=[.001, .005, .05, .5] J/K  thermal_time_constant=[.001, .2] s  thermal_time_constant_Cauer=[.001, .1, .2] s  thermal_time_constant_Foster=[7e-05, .0007, .01, .08] s  thermal_mass_initial_temperatures=[25, 25] degC  thermal_mass_initial_temperatures_Cauer=[25, 25, 25] degC  junction_thermal_mass=0.01 J/K  Tvec_initial_Foster=[25, 25, 25, 25] degC  junction_temperature_specify=off  junction_temperature_priority=None  junction_temperature=25 degC  junction_temperature_nominal_specify=off  junction_temperature_nominal_value=1  junction_temperature_nominal_unit=degC  Qj_specify=off  Qj_priority=None  Qj=0 W  Qj_nominal_specify=off  Qj_nominal_value=1  Qj_nominal_unit=W  accumulatedSwitchingLosses_specify=off  accumulatedSwitchingLosses_priority=None  accumulatedSwitchingLosses=0 J
      settings: InternalSimscapePortConfiguration="{\"Bottom\":[],\"Left\":[{\"id\":\"G\",\"label\":\"\",\"type\":\"input\"}],\"Right\":[{\"id\":\"A\",\"label\":\"\",\"type\":\"foundation.electrical.electrical\"},{\"id\":\"K\",\"label\":\"\",\"type\":\"foundation.electrical.electrical\"}],\"Top\":[]}"
  firing1 : Subsystem
  firing2 : Subsystem
  firing3 : Subsystem
  firing4 : Subsystem
  firing5 : Subsystem
  firing6 : Subsystem
  snubber_{1..6} (6 alike) : fl_lib/Electrical/Electrical Elements/Capacitor  c=Csnubber_scr F  r=Rsnubber_scr Ohm  g=0 1/Ohm  i_specify=off  i_priority=None  i=0 A  i_nominal_specify=off  i_nominal_value=1  i_nominal_unit=A  v_specify=off  v_priority=None  v=0 V  v_nominal_specify=off  v_nominal_value=1  v_nominal_unit=V  vc_specify=off  vc_priority=High  vc=0 V  vc_nominal_specify=off  vc_nominal_value=1  vc_nominal_unit=V
  DC+ : PMIOPort  Side=Left
  G1 : PMIOPort  Port=2  Side=Left
  G2 : PMIOPort  Port=3  Side=Left
  G3 : PMIOPort  Port=4  Side=Left
  G4 : PMIOPort  Port=5  Side=Left
  G5 : PMIOPort  Port=6  Side=Left
  G6 : PMIOPort  Port=7  Side=Left
  DC- : PMIOPort  Port=8  Side=Left
  phA : PMIOPort  Port=9  Side=Right
  phB : PMIOPort  Port=10  Side=Right
  phC : PMIOPort  Port=11  Side=Right
  connections:
  DC+/RConn1 -- snubber_5/LConn1 -- T5/RConn2 -- snubber_3/LConn1 -- T3/RConn2 -- snubber_1/LConn1 -- T1/RConn2
  T1/RConn1 -- snubber_1/RConn1 -- snubber_4/LConn1 -- T4/RConn2 -- phA/RConn1
  T2/RConn2 -- snubber_2/LConn1 -- snubber_5/RConn1 -- T5/RConn1 -- phC/RConn1
  T3/RConn1 -- snubber_3/RConn1 -- snubber_6/LConn1 -- T6/RConn2 -- phB/RConn1
  T2/RConn1 -- snubber_2/RConn1 -- snubber_6/RConn1 -- T6/RConn1 -- snubber_4/RConn1 -- T4/RConn1 -- DC-/RConn1
  G1/RConn1 -- firing1/LConn1
  G2/RConn1 -- firing2/LConn1
  G3/RConn1 -- firing3/LConn1
  G4/RConn1 -- firing4/LConn1
  G5/RConn1 -- firing5/LConn1
  G6/RConn1 -- firing6/LConn1
  firing1/RConn1 -- T1/LConn1
  firing2/RConn1 -- T2/LConn1
  firing3/RConn1 -- T3/LConn1
  firing4/RConn1 -- T4/LConn1
  firing5/RConn1 -- T5/LConn1
  firing6/RConn1 -- T6/LConn1

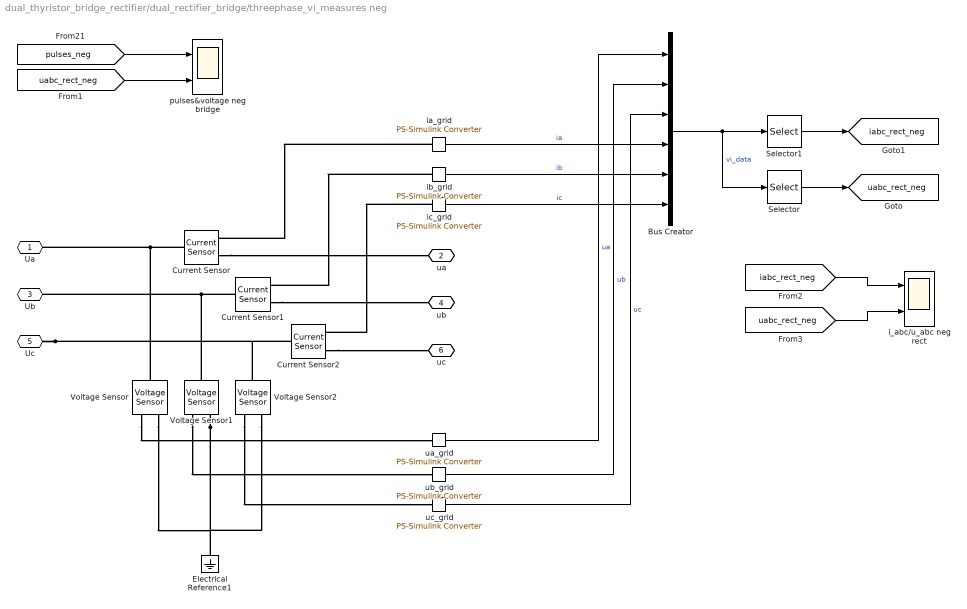
== system dual_thyristor_bridge_rectifier/dual_rectifier_bridge/threephase_vi_measures neg ==
  Bus Creator : BusCreator  Inputs=6
  Current Sensor : fl_lib/Electrical/Electrical Sensors/Current Sensor
  Current Sensor1 : fl_lib/Electrical/Electrical Sensors/Current Sensor
  Current Sensor2 : fl_lib/Electrical/Electrical Sensors/Current Sensor
  Electrical Reference1 : fl_lib/Electrical/Electrical Elements/Electrical Reference
  Selector : Selector  InputPortWidth=6  IndexOptions=Index vector (dialog)  Indices=[1 2 3]  OutputSizes=1
  Selector1 : Selector  InputPortWidth=6  IndexOptions=Index vector (dialog)  Indices=[4 5 6]  OutputSizes=1
  Voltage Sensor : fl_lib/Electrical/Electrical Sensors/Voltage Sensor
  Voltage Sensor1 : fl_lib/Electrical/Electrical Sensors/Voltage Sensor
  Voltage Sensor2 : fl_lib/Electrical/Electrical Sensors/Voltage Sensor
  i_abc/u_abc neg rect : Scope  NumInputPorts=2
      settings: SampleTime=tc  ActiveDisplayYMinimum=-1644.00062  ActiveDisplayYMaximum=1640.15476  DataLoggingVariableName=ScopeData2
  ia_grid : nesl_utility/PS-Simulink Converter  PhysicalDomain=network_engine_domain  SubClassName=ps_output  LeftPortType=input  RightPortType=output  PseudoPeriodic=off  Frequencies=[]  VectorFormat=1-D array  Unit=A  AffineConversion=off
  ib_grid : nesl_utility/PS-Simulink Converter  PhysicalDomain=network_engine_domain  SubClassName=ps_output  LeftPortType=input  RightPortType=output  PseudoPeriodic=off  Frequencies=[]  VectorFormat=1-D array  Unit=A  AffineConversion=off
  ic_grid : nesl_utility/PS-Simulink Converter  PhysicalDomain=network_engine_domain  SubClassName=ps_output  LeftPortType=input  RightPortType=output  PseudoPeriodic=off  Frequencies=[]  VectorFormat=1-D array  Unit=A  AffineConversion=off
  pulses&voltage neg bridge : Scope  NumInputPorts=2
      settings: SampleTime=tc  ActiveDisplayYMinimum=-1644.00062  ActiveDisplayYMaximum=1640.15476  DataLoggingVariableName=ScopeData2
  ua_grid : nesl_utility/PS-Simulink Converter  PhysicalDomain=network_engine_domain  SubClassName=ps_output  LeftPortType=input  RightPortType=output  PseudoPeriodic=off  Frequencies=[]  VectorFormat=1-D array  Unit=V  AffineConversion=off
  ub_grid : nesl_utility/PS-Simulink Converter  PhysicalDomain=network_engine_domain  SubClassName=ps_output  LeftPortType=input  RightPortType=output  PseudoPeriodic=off  Frequencies=[]  VectorFormat=1-D array  Unit=V  AffineConversion=off
  uc_grid : nesl_utility/PS-Simulink Converter  PhysicalDomain=network_engine_domain  SubClassName=ps_output  LeftPortType=input  RightPortType=output  PseudoPeriodic=off  Frequencies=[]  VectorFormat=1-D array  Unit=V  AffineConversion=off
  Ua : PMIOPort  Side=Left
  ua : PMIOPort  Port=2  Side=Right
  Ub : PMIOPort  Port=3  Side=Left
  ub : PMIOPort  Port=4  Side=Right
  Uc : PMIOPort  Port=5  Side=Left
  uc : PMIOPort  Port=6  Side=Right
  tag scope: iabc_rect_neg=global, uabc_rect_neg=global
  wires:
  [iabc_rect_neg] -> i_abc/u_abc neg rect/1
  [uabc_rect_neg] -> i_abc/u_abc neg rect/2
  Selector1/1 -> [iabc_rect_neg]
  uc_grid/1 -> Bus Creator/3  "uc"
  ub_grid/1 -> Bus Creator/2  "ub"
  ua_grid/1 -> Bus Creator/1  "ua"
  ic_grid/1 -> Bus Creator/6  "ic"
  ia_grid/1 -> Bus Creator/4  "ia"
  ib_grid/1 -> Bus Creator/5  "ib"
  Selector/1 -> [uabc_rect_neg]
  Bus Creator/1 -> Selector/1, Selector1/1  "vi_data"
  [pulses_neg] -> pulses&voltage neg bridge/1
  [uabc_rect_neg] -> pulses&voltage neg bridge/2
  connections:
  Current Sensor2/RConn2 -- uc/RConn1
  ic_grid/LConn1 -- Current Sensor2/RConn1
  ia_grid/LConn1 -- Current Sensor/RConn1
  ib_grid/LConn1 -- Current Sensor1/RConn1
  Voltage Sensor2/RConn1 -- uc_grid/LConn1
  Current Sensor1/RConn2 -- ub/RConn1
  Voltage Sensor/LConn1 -- Ua/RConn1 -- Current Sensor/LConn1
  Uc/RConn1 -- Current Sensor2/LConn1 -- Voltage Sensor2/LConn1
  Voltage Sensor1/RConn1 -- ub_grid/LConn1
  Current Sensor/RConn2 -- ua/RConn1
  Voltage Sensor/RConn1 -- ua_grid/LConn1
  Voltage Sensor1/RConn2 -- Voltage Sensor2/RConn2 -- Voltage Sensor/RConn2 -- Electrical Reference1/LConn1
  Voltage Sensor1/LConn1 -- Ub/RConn1 -- Current Sensor1/LConn1

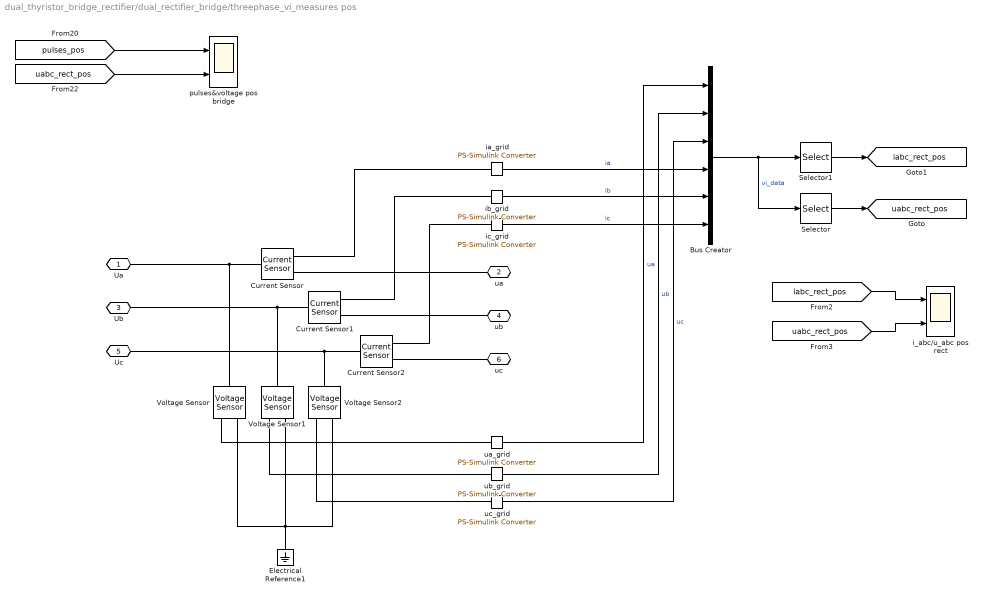
== system dual_thyristor_bridge_rectifier/dual_rectifier_bridge/threephase_vi_measures pos ==
  Bus Creator : BusCreator  Inputs=6
  Current Sensor : fl_lib/Electrical/Electrical Sensors/Current Sensor
  Current Sensor1 : fl_lib/Electrical/Electrical Sensors/Current Sensor
  Current Sensor2 : fl_lib/Electrical/Electrical Sensors/Current Sensor
  Electrical Reference1 : fl_lib/Electrical/Electrical Elements/Electrical Reference
  Selector : Selector  InputPortWidth=6  IndexOptions=Index vector (dialog)  Indices=[1 2 3]  OutputSizes=1
  Selector1 : Selector  InputPortWidth=6  IndexOptions=Index vector (dialog)  Indices=[4 5 6]  OutputSizes=1
  Voltage Sensor : fl_lib/Electrical/Electrical Sensors/Voltage Sensor
  Voltage Sensor1 : fl_lib/Electrical/Electrical Sensors/Voltage Sensor
  Voltage Sensor2 : fl_lib/Electrical/Electrical Sensors/Voltage Sensor
  i_abc/u_abc pos rect : Scope  NumInputPorts=2
      settings: SampleTime=tc  ActiveDisplayYMinimum=-3631.80998  ActiveDisplayYMaximum=3630.93687  DataLoggingVariableName=ScopeData2
  ia_grid : nesl_utility/PS-Simulink Converter  PhysicalDomain=network_engine_domain  SubClassName=ps_output  LeftPortType=input  RightPortType=output  PseudoPeriodic=off  Frequencies=[]  VectorFormat=1-D array  Unit=A  AffineConversion=off
  ib_grid : nesl_utility/PS-Simulink Converter  PhysicalDomain=network_engine_domain  SubClassName=ps_output  LeftPortType=input  RightPortType=output  PseudoPeriodic=off  Frequencies=[]  VectorFormat=1-D array  Unit=A  AffineConversion=off
  ic_grid : nesl_utility/PS-Simulink Converter  PhysicalDomain=network_engine_domain  SubClassName=ps_output  LeftPortType=input  RightPortType=output  PseudoPeriodic=off  Frequencies=[]  VectorFormat=1-D array  Unit=A  AffineConversion=off
  pulses&voltage pos bridge : Scope  NumInputPorts=2
      settings: SampleTime=tc  ActiveDisplayYMinimum=-0.125  ActiveDisplayYMaximum=1.125
  ua_grid : nesl_utility/PS-Simulink Converter  PhysicalDomain=network_engine_domain  SubClassName=ps_output  LeftPortType=input  RightPortType=output  PseudoPeriodic=off  Frequencies=[]  VectorFormat=1-D array  Unit=V  AffineConversion=off
  ub_grid : nesl_utility/PS-Simulink Converter  PhysicalDomain=network_engine_domain  SubClassName=ps_output  LeftPortType=input  RightPortType=output  PseudoPeriodic=off  Frequencies=[]  VectorFormat=1-D array  Unit=V  AffineConversion=off
  uc_grid : nesl_utility/PS-Simulink Converter  PhysicalDomain=network_engine_domain  SubClassName=ps_output  LeftPortType=input  RightPortType=output  PseudoPeriodic=off  Frequencies=[]  VectorFormat=1-D array  Unit=V  AffineConversion=off
  Ua : PMIOPort  Side=Left
  ua : PMIOPort  Port=2  Side=Right
  Ub : PMIOPort  Port=3  Side=Left
  ub : PMIOPort  Port=4  Side=Right
  Uc : PMIOPort  Port=5  Side=Left
  uc : PMIOPort  Port=6  Side=Right
  tag scope: iabc_rect_pos=global, uabc_rect_pos=global
  wires:
  Bus Creator/1 -> Selector1/1, Selector/1  "vi_data"
  Selector/1 -> [uabc_rect_pos]
  ib_grid/1 -> Bus Creator/5  "ib"
  ia_grid/1 -> Bus Creator/4  "ia"
  ic_grid/1 -> Bus Creator/6  "ic"
  ua_grid/1 -> Bus Creator/1  "ua"
  ub_grid/1 -> Bus Creator/2  "ub"
  uc_grid/1 -> Bus Creator/3  "uc"
  Selector1/1 -> [iabc_rect_pos]
  [uabc_rect_pos] -> i_abc/u_abc pos rect/2
  [iabc_rect_pos] -> i_abc/u_abc pos rect/1
  [pulses_pos] -> pulses&voltage pos bridge/1
  [uabc_rect_pos] -> pulses&voltage pos bridge/2
  connections:
  Current Sensor1/LConn1 -- Ub/RConn1 -- Voltage Sensor1/LConn1
  Electrical Reference1/LConn1 -- Voltage Sensor/RConn2 -- Voltage Sensor2/RConn2 -- Voltage Sensor1/RConn2
  Voltage Sensor/RConn1 -- ua_grid/LConn1
  Current Sensor/RConn2 -- ua/RConn1
  Voltage Sensor1/RConn1 -- ub_grid/LConn1
  Voltage Sensor2/LConn1 -- Current Sensor2/LConn1 -- Uc/RConn1
  Current Sensor/LConn1 -- Ua/RConn1 -- Voltage Sensor/LConn1
  Current Sensor1/RConn2 -- ub/RConn1
  Voltage Sensor2/RConn1 -- uc_grid/LConn1
  ib_grid/LConn1 -- Current Sensor1/RConn1
  ia_grid/LConn1 -- Current Sensor/RConn1
  ic_grid/LConn1 -- Current Sensor2/RConn1
  Current Sensor2/RConn2 -- uc/RConn1
